simulink model "RescueBot_Full_System"  (R2025b)
settings: Solver=VariableStepAuto  StartTime=0.0  StopTime=10.0  RelTol=1e-3
settings Model: Creator=palellabhanuprasad  LastModifiedBy=palellabhanuprasad

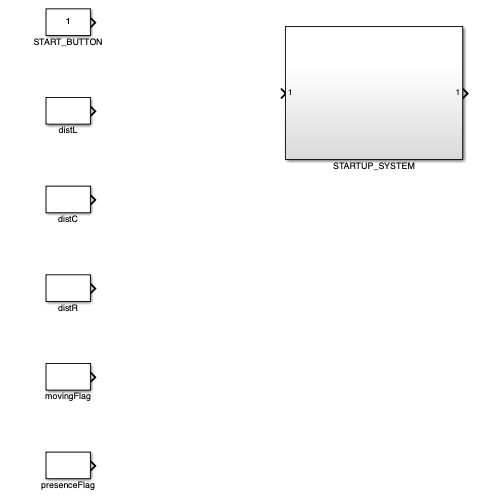
[thumbnail: Simulink's stored preview of the top-level diagram]
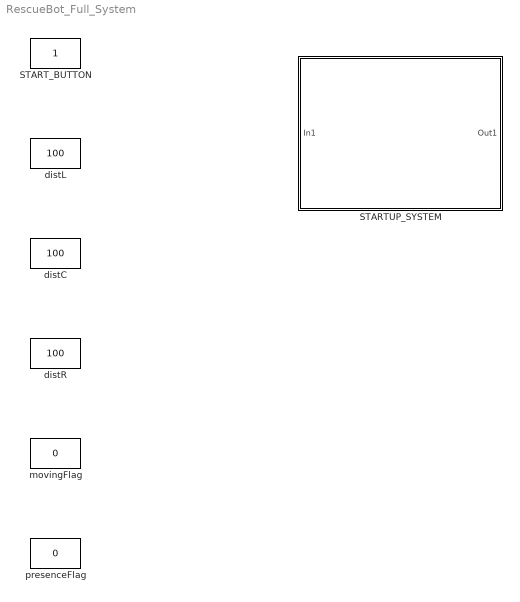
== system RescueBot_Full_System ==
  STARTUP_SYSTEM : Subsystem
  START_BUTTON : Constant
  distC : Constant  Value=100
  distL : Constant  Value=100
  distR : Constant  Value=100
  movingFlag : Constant  Value=0
  presenceFlag : Constant  Value=0

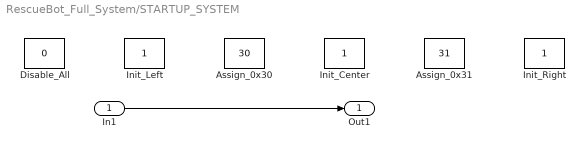
== system RescueBot_Full_System/STARTUP_SYSTEM ==
  In1 : Inport
  Assign_0x30 : Constant  Value=30
  Assign_0x31 : Constant  Value=31
  Disable_All : Constant  Value=0
  Init_Center : Constant
  Init_Left : Constant
  Init_Right : Constant
  Out1 : Outport
  wires:
  In1/1 -> Out1/1
